simulink library "wheel_loader_contact_lib"  (R2025a)
settings: Solver=VariableStepAuto  StartTime=0.0  StopTime=10.0  RelTol=1e-3
undefined symbols (not defined in the file): HMPST, ptcld, X, Y, Z
libraries: sm_lib x11, nesl_utility x2, grid_element x1
Description:
  | Copyright 2023-2025 The MathWorks, Inc.
settings Model: Creator=smiller  LastModifiedBy=smiller
settings RTWCC: GPUComputeCapability=3.5

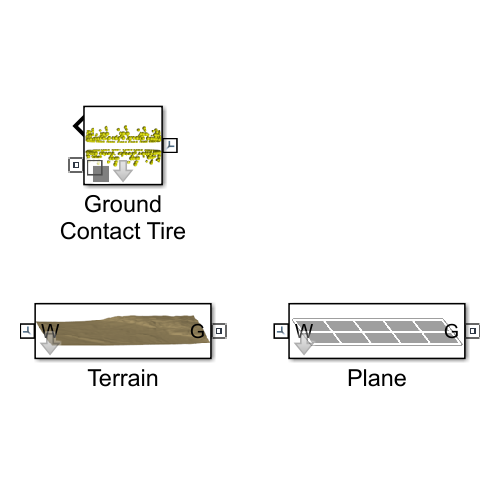
[thumbnail: Simulink's stored preview of the top-level diagram]
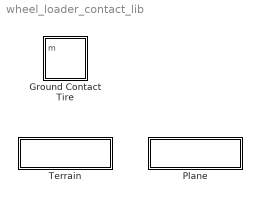
== system wheel_loader_contact_lib ==
  Ground Contact Tire : Subsystem  Variant=on  VariantControlMode=label  VariantControl=Choice  LabelModeActiveChoice=Points  mask{popup_contact=Points, ptcld_xyz=ptcld.LR}
      mask prompts: popup_contact "Contact Geometry"; ptcld_xyz "Point Cloud [x y z] (mm)"
      mask init:
      | contactChoice = get_param(gcb,'popup_contact');
      | set_param(gcb,'LabelModeActiveChoice',contactChoice)
      | %if(popup_contact == 1)
      | %    set_param(gcb,'LabelModeActiveChoice','Sphere')
      | %elseif(popup_contact == 2)
      | %    set_param(gcb,'LabelModeActiveChoice','Points')
      | %elseif(popup_contact == 3)
      | %    set_param(gcb,'LabelModeActiveChoice','Tire')
      | %end
      mask TypeOptions popup_contact: Sphere | Points | Tire
  Plane : Subsystem  VariantControl=Plane
      mask Display: image('sm_wheel_loader_tire_surface_plane_IMAGE.png');
  Terrain : Subsystem
      mask Display: image('sm_wheel_loader_tire_surface_terrain_IMAGE.png')

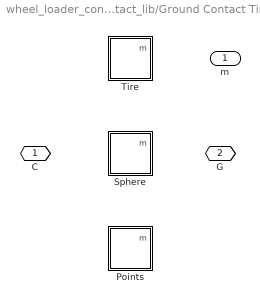
== system wheel_loader_contact_lib/Ground Contact Tire ==
  Points : Subsystem  VariantControl=Points  mask{CoordinatesMatrix=ptcld_xyz}
      mask prompts: CoordinatesMatrix "Points [x y z] (mm)"
      mask TypeOptions CoordinatesMatrix: Point Cloud/CoordinatesMatrix
      mask Display: image('sm_wheel_loader_tire_contact_points_IMAGE.png')
  Sphere : Subsystem  VariantControl=Sphere
      mask Display: image('sm_wheel_loader_tire_contact_sphere_IMAGE.png')
  Tire : Subsystem  VariantControl=Tire
      mask Display: image('sm_wheel_loader_tire_contact_magicFormula_IMAGE.png')
  C : PMIOPort  Side=Left
  G : PMIOPort  Port=2  Side=Right
  m : Outport

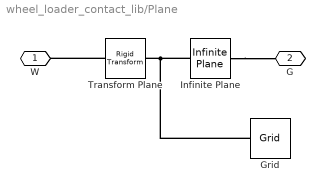
== system wheel_loader_contact_lib/Plane ==
  Grid : grid_element/Grid  VariantControl=Grid  grid_x=16  grid_y=12  grid_z=0.02  grid_line_width=0.02  grid_num_sq_x=4*2  grid_num_sq_y=3*2  grid_clr=[1 1 1]  plane_clr=[1 1 1]  grid_opc=1  plane_opc=1
  Infinite Plane : sm_lib/Curves and Surfaces/Infinite Plane  GraphicType=Rectangle  GraphicPlaneWidth=16  GraphicPlaneWidthUnits=mm  GraphicPlaneHeight=12  GraphicPlaneHeightUnits=mm  GraphicVisPropType=SimpleVisualProperties  GraphicDiffuseColor=[1 1 1]  GraphicOpacity=0  GraphicSpecularColor=[0.5 0.5 0.5 1.0]  GraphicAmbientColor=[0.15 0.15 0.15 1.0]  GraphicEmissiveColor=[0.0 0.0 0.0 1.0]  GraphicShininess=75
  Transform Plane : sm_lib/Frames and Transforms/Rigid Transform  RotationMethod=None  FollAlignAxisA=+X  BaseAlignAxisA=+Y  FollAlignAxisB=+Y  BaseAlignAxisB=+Z  RotationStandardAxis=+Z  RotationAngle=0.0  RotationAngleUnits=deg  RotationArbitraryAxis=[0 0 1]  RotationSequenceAxes=FollowerAxes  RotationSequence=XYX  RotationSequenceAngles=[0 0 0]  RotationSequenceAnglesUnits=deg  RotationMatrix=[1 0 0; 0 1 0; 0 0 1]  Quaternion=[1 0 0 0]  TranslationMethod=Cartesian  TranslationCartesianOffset=[0 -3500+870.5 0]  TranslationCartesianOffsetUnits=mm  TranslationStandardAxis=+Z  TranslationStandardOffset=0  TranslationStandardOffsetUnits=m  TranslationROffset=0  TranslationROffsetUnits=m  TranslationThetaOffset=0  TranslationThetaOffsetUnits=deg  TranslationZOffset=0  TranslationZOffsetUnits=m
  W : PMIOPort  Side=Left
  G : PMIOPort  Port=2  Side=Right
  connections:
  Transform Plane/LConn1 -- W/RConn1
  Infinite Plane/RConn1 -- G/RConn1
  Transform Plane/RConn1 -- Infinite Plane/LConn1 -- Grid/RConn1

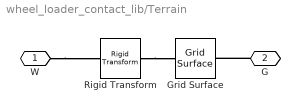
== system wheel_loader_contact_lib/Terrain ==
  Grid Surface : sm_lib/Curves and Surfaces/Grid Surface  XGridVector=Scene.Terrain.xg  XGridVectorUnits=m  YGridVector=Scene.Terrain.yg  YGridVectorUnits=m  ZHeights=Scene.Terrain.z_heights_data  ZHeightsUnits=m  GraphicType=FromGeometry  GraphicVisPropType=SimpleVisualProperties  GraphicDiffuseColor=[0.8196 0.7255 0.5098]  GraphicOpacity=1.0  GraphicSpecularColor=[0.5 0.5 0.5 1.0]  GraphicAmbientColor=[0.15 0.15 0.15 1.0]  GraphicEmissiveColor=[0.0 0.0 0.0 1.0]  GraphicShininess=75
  Rigid Transform : sm_lib/Frames and Transforms/Rigid Transform  RotationMethod=None  FollAlignAxisA=+X  BaseAlignAxisA=+Y  FollAlignAxisB=+Y  BaseAlignAxisB=+Z  RotationStandardAxis=+Z  RotationAngle=0.0  RotationAngleUnits=deg  RotationArbitraryAxis=[0 0 1]  RotationSequenceAxes=FollowerAxes  RotationSequence=XYX  RotationSequenceAngles=[0 0 0]  RotationSequenceAnglesUnits=deg  RotationMatrix=[1 0 0; 0 1 0; 0 0 1]  Quaternion=[1 0 0 0]  TranslationMethod=Cartesian  TranslationCartesianOffset=[-20 -32 -1.3]  TranslationCartesianOffsetUnits=m  TranslationStandardAxis=+Z  TranslationStandardOffset=0  TranslationStandardOffsetUnits=m  TranslationROffset=0  TranslationROffsetUnits=m  TranslationThetaOffset=0  TranslationThetaOffsetUnits=deg  TranslationZOffset=0  TranslationZOffsetUnits=m
  W : PMIOPort  Side=Left
  G : PMIOPort  Port=2  Side=Right
  connections:
  W/RConn1 -- Rigid Transform/LConn1
  Rigid Transform/RConn1 -- Grid Surface/LConn1
  G/RConn1 -- Grid Surface/RConn1

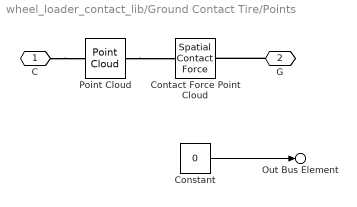
== system wheel_loader_contact_lib/Ground Contact Tire/Points ==
  Constant : Constant  Value=0
  Contact Force Point Cloud : sm_lib/Forces and Torques/Spatial Contact Force  SenseSeparationDistance=off  NormalForceType=SmoothSpringDamper  NormalStiffness=HMPST.Tire.Contact.ptcld.stiffness  NormalStiffnessUnits=N/m  NormalDamping=HMPST.Tire.Contact.ptcld.damping  NormalDampingUnits=N/(m/s)  NormalTransitionRegionWidth=HMPST.Tire.Contact.ptcld.transRegWidth  NormalTransitionRegionWidthUnits=m  FrictionType=SmoothStickSlip  CoefficientOfStaticFriction=HMPST.Tire.Contact.ptcld.muStatic  CoefficientOfDynamicFriction=HMPST.Tire.Contact.ptcld.muDynamic  FrictionalCriticalVelocity=HMPST.Tire.Contact.ptcld.velThreshold  FrictionalCriticalVelocityUnits=m/s  SenseContactSignal=off  SensePenetrationDepth=off  SenseNormalVelocity=off  SenseTangentialVelocity=off  SensingForceTorqueDirection=BaseOnFollower  SensingForceTorqueResolutionFrame=ContactFrame  SenseNormalForce=off  SenseNormalForceMagnitude=off  SenseNormalTorque=off  SenseFrictionalForce=off  SenseFrictionalForceMagnitude=off  SenseFrictionalTorque=off  SenseTotalForce=off  SenseTotalTorque=off  SenseContactBaseRotation=off  SenseContactBaseTranslation=off  SenseContactFollowerRotation=off  SenseContactFollowerTranslation=off  ZeroCrossDetectContactStartAndEnd=off
  Point Cloud : sm_lib/Curves and Surfaces/Point Cloud  CoordinatesMatrix=CoordinatesMatrix  CoordinatesMatrixUnits=mm  GraphicType=MarkerCloud  GraphicSphereRadius=5e-3  GraphicSphereRadiusUnits=m  GraphicVisPropType=SimpleVisualProperties  GraphicDiffuseColor=[1 1 0.06667]  GraphicOpacity=1.0  GraphicSpecularColor=[0.5 0.5 0.5 1.0]  GraphicAmbientColor=[0.15 0.15 0.15 1.0]  GraphicEmissiveColor=[0.0 0.0 0.0 1.0]  GraphicShininess=75
  C : PMIOPort  Side=Left
  G : PMIOPort  Port=2  Side=Right
  Out Bus Element : Outport  PortName=m  Element=Fn
  wires:
  Constant/1 -> Out Bus Element/1
  connections:
  G/RConn1 -- Contact Force Point Cloud/LConn1
  Point Cloud/RConn1 -- Contact Force Point Cloud/RConn1
  C/RConn1 -- Point Cloud/LConn1

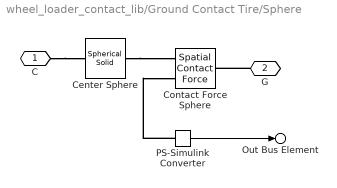
== system wheel_loader_contact_lib/Ground Contact Tire/Sphere ==
  Center Sphere : sm_lib/Body Elements/Spherical Solid  SphereRadius=HMPST.Tire.Rad  SphereRadiusUnits=m  ExportEntireGeometry=on  InertiaType=CalculateFromGeometry  BasedOnType=Density  Density=1  DensityUnits=kg/m^3  Mass=1  MassUnits=kg  CenterOfMass=[0 0 0]  CenterOfMassUnits=m  MomentsOfInertia=[1 1 1]  MomentsOfInertiaUnits=kg*m^2  ProductsOfInertia=[0 0 0]  ProductsOfInertiaUnits=kg*m^2  GraphicType=None  MarkerShape=Sphere  MarkerSize=10  GraphicVisPropType=SimpleVisualProperties  GraphicDiffuseColor=[0.5 0.5 0.5]  GraphicOpacity=0.5  GraphicSpecularColor=[0.5 0.5 0.5 1.0]  GraphicAmbientColor=[0.15 0.15 0.15 1.0]  GraphicEmissiveColor=[0.0 0.0 0.0 1.0]  GraphicShininess=75  DoExposeReferenceFrame=on  SerializedFrames=<Frames/>
  Contact Force Sphere : sm_lib/Forces and Torques/Spatial Contact Force  SenseSeparationDistance=off  NormalForceType=SmoothSpringDamper  NormalStiffness=HMPST.Tire.Contact.sphere.stiffness  NormalStiffnessUnits=N/m  NormalDamping=HMPST.Tire.Contact.sphere.damping  NormalDampingUnits=N/(m/s)  NormalTransitionRegionWidth=HMPST.Tire.Contact.sphere.transRegWidth  NormalTransitionRegionWidthUnits=m  FrictionType=SmoothStickSlip  CoefficientOfStaticFriction=HMPST.Tire.Contact.sphere.muStatic  CoefficientOfDynamicFriction=HMPST.Tire.Contact.sphere.muDynamic  FrictionalCriticalVelocity=HMPST.Tire.Contact.sphere.velThreshold  FrictionalCriticalVelocityUnits=m/s  SenseContactSignal=off  SensePenetrationDepth=off  SenseNormalVelocity=off  SenseTangentialVelocity=off  SensingForceTorqueDirection=BaseOnFollower  SensingForceTorqueResolutionFrame=ContactFrame  SenseNormalForce=off  SenseNormalForceMagnitude=on  SenseNormalTorque=off  SenseFrictionalForce=off  SenseFrictionalForceMagnitude=off  SenseFrictionalTorque=off  SenseTotalForce=off  SenseTotalTorque=off  SenseContactBaseRotation=off  SenseContactBaseTranslation=off  SenseContactFollowerRotation=off  SenseContactFollowerTranslation=off  ZeroCrossDetectContactStartAndEnd=off
  PS-Simulink Converter : nesl_utility/PS-Simulink Converter  PhysicalDomain=network_engine_domain  SubClassName=ps_output  LeftPortType=input  RightPortType=output  PseudoPeriodic=off  Frequencies=[]  VectorFormat=inherit  Unit=inherit  AffineConversion=off
  C : PMIOPort  Side=Left
  G : PMIOPort  Port=2  Side=Right
  Out Bus Element : Outport  PortName=m  Element=Fn
  wires:
  PS-Simulink Converter/1 -> Out Bus Element/1
  connections:
  Center Sphere/LConn1 -- Contact Force Sphere/RConn1
  C/RConn1 -- Center Sphere/RConn1
  G/RConn1 -- Contact Force Sphere/LConn1
  PS-Simulink Converter/LConn1 -- Contact Force Sphere/RConn2

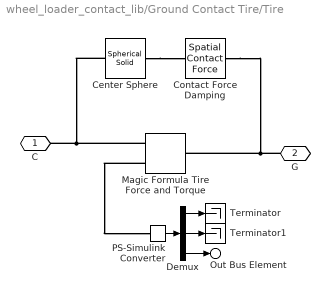
== system wheel_loader_contact_lib/Ground Contact Tire/Tire ==
  Center Sphere : sm_lib/Body Elements/Spherical Solid  SphereRadius=HMPST.Tire.Rad  SphereRadiusUnits=m  ExportEntireGeometry=on  InertiaType=CalculateFromGeometry  BasedOnType=Density  Density=1  DensityUnits=kg/m^3  Mass=1  MassUnits=kg  CenterOfMass=[0 0 0]  CenterOfMassUnits=m  MomentsOfInertia=[1 1 1]  MomentsOfInertiaUnits=kg*m^2  ProductsOfInertia=[0 0 0]  ProductsOfInertiaUnits=kg*m^2  GraphicType=None  MarkerShape=Sphere  MarkerSize=10  GraphicVisPropType=SimpleVisualProperties  GraphicDiffuseColor=[0.5 0.5 0.5]  GraphicOpacity=0.5  GraphicSpecularColor=[0.5 0.5 0.5 1.0]  GraphicAmbientColor=[0.15 0.15 0.15 1.0]  GraphicEmissiveColor=[0.0 0.0 0.0 1.0]  GraphicShininess=75  DoExposeReferenceFrame=on  SerializedFrames=<Frames/>
  Contact Force Damping : sm_lib/Forces and Torques/Spatial Contact Force  SenseSeparationDistance=off  NormalForceType=SmoothSpringDamper  NormalStiffness=HMPST.Tire.Contact.sphere.stiffness*0  NormalStiffnessUnits=N/m  NormalDamping=HMPST.Tire.Contact.sphere.damping  NormalDampingUnits=N/(m/s)  NormalTransitionRegionWidth=HMPST.Tire.Contact.sphere.transRegWidth  NormalTransitionRegionWidthUnits=m  FrictionType=None  CoefficientOfStaticFriction=HMPST.Tire.Contact.sphere.muStatic  CoefficientOfDynamicFriction=HMPST.Tire.Contact.sphere.muDynamic  FrictionalCriticalVelocity=HMPST.Tire.Contact.sphere.velThreshold  FrictionalCriticalVelocityUnits=m/s  SenseContactSignal=off  SensePenetrationDepth=off  SenseNormalVelocity=off  SenseTangentialVelocity=off  SensingForceTorqueDirection=BaseOnFollower  SensingForceTorqueResolutionFrame=ContactFrame  SenseNormalForce=off  SenseNormalForceMagnitude=off  SenseNormalTorque=off  SenseFrictionalForce=off  SenseFrictionalForceMagnitude=off  SenseFrictionalTorque=off  SenseTotalForce=off  SenseTotalTorque=off  SenseContactBaseRotation=off  SenseContactBaseTranslation=off  SenseContactFollowerRotation=off  SenseContactFollowerTranslation=off  ZeroCrossDetectContactStartAndEnd=off
  Demux : Demux  Outputs=3
  Magic Formula Tire Force and Torque : sm_lib/Forces and Torques/Magic Formula Tire Force and Torque  TireSide=Left  TireParameters=HMPST.Tire.Contact  SlipMode=Combined  ContactFrameMethod=ClosestPoint  ScalingCoefficientLMUXMode=FromTireParameters  ScalingCoefficientLMUYMode=FromTireParameters  SenseContactSignal=off  TireWrenchFrame=ContactFrame  SenseTireForce=on  SenseTireTorque=off  SensePneumaticTrail=off  SenseLongitudinalSlip=off  SenseSaturatedLongitudinalSlip=off  SenseSlipAngle=off  SenseSaturatedSlipAngle=off  SenseTurnSlip=off  SenseRelativeLongitudinalVelocity=off  SenseRelativeLateralVelocity=off  SenseLongitudinalSlipVelocity=off  SenseLateralSlipVelocity=off  SenseYawVelocity=off  SenseCamberAngle=off  SenseSaturatedCamberAngle=off  SenseCamberVelocity=off  SenseSpinVelocity=off  SenseFreeRadius=off  SenseLoadedRadius=off  SenseEffectiveRollingRadius=off  SenseRadialDeflection=off  SenseLongitudinalFrictionCoefficient=off  SenseLateralFrictionCoefficient=off  SenseContactBaseRotation=off  SenseContactBaseTranslation=off  SenseContactFollowerRotation=off  SenseContactFollowerTranslation=off  NumericParameters=[0.1 0.1 0.1 0.1 5.0 1e-4 1e-4 1e-7 1e-7 1e-4 1e-4 0.1 1e-4 1e-4 1e-4 1e-4 1e-4 1e-4 1e-4 1e-4 1e-4]
  PS-Simulink Converter : nesl_utility/PS-Simulink Converter  PhysicalDomain=network_engine_domain  SubClassName=ps_output  LeftPortType=input  RightPortType=output  PseudoPeriodic=off  Frequencies=[]  VectorFormat=inherit  Unit=inherit  AffineConversion=off
  Terminator : Terminator
  Terminator1 : Terminator
  C : PMIOPort  Side=Left
  G : PMIOPort  Port=2  Side=Right
  Out Bus Element : Outport  PortName=m  Element=Fn
  wires:
  PS-Simulink Converter/1 -> Demux/1
  Demux/3 -> Out Bus Element/1
  Demux/1 -> Terminator/1
  Demux/2 -> Terminator1/1
  connections:
  G/RConn1 -- Contact Force Damping/LConn1 -- Magic Formula Tire Force and Torque/LConn1
  Magic Formula Tire Force and Torque/RConn1 -- Center Sphere/RConn1 -- C/RConn1
  Magic Formula Tire Force and Torque/RConn2 -- PS-Simulink Converter/LConn1
  Center Sphere/LConn1 -- Contact Force Damping/RConn1
